simulink model "BMS_Protection_SoC"  (R2026b)
settings: Solver=VariableStepAuto
libraries: simulink x2
settings Model: Creator=maryliya  LastModifiedBy=maryliya

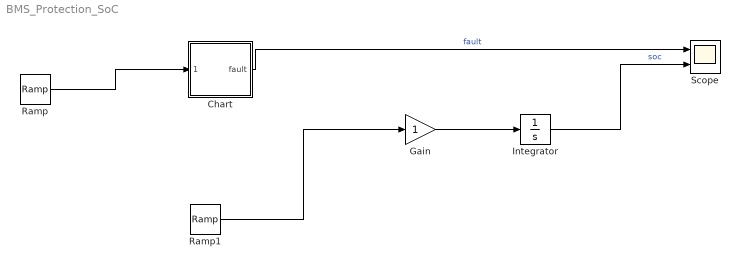
== system BMS_Protection_SoC ==
  Chart : Stateflow chart  TreatAsAtomicUnit=on
  Gain : Gain
  Integrator : Integrator
  Ramp : simulink/Sources/Ramp  slope=0.2  start=0  InitialOutput=2.8
  Ramp1 : simulink/Sources/Ramp  slope=1  start=0  InitialOutput=0
  Scope : Scope  NumInputPorts=2
      settings: ActiveDisplayYMinimum=-6.2500000000000027  ActiveDisplayYMaximum=56.250000000000043
  wires:
  Ramp1/1 -> Gain/1
  Gain/1 -> Integrator/1
  Ramp/1 -> Chart/1(voltage)
  Integrator/1 -> Scope/2  "soc"
  Chart/1(fault) -> Scope/1  "fault"

== stateflow chart BMS_Protection_SoC/Chart ==
  state Normal
    fault=0
  state OverVoltage_Fault
    fault=1
  state UnderVoltage_Fault
    fault=2
  Normal -> OverVoltage_Fault [order 1] : [voltage>4.2]
  OverVoltage_Fault -> Normal : [voltage<=4.2]
  (default) -> Normal
  Normal -> UnderVoltage_Fault [order 2] : [voltage<3.0]
  UnderVoltage_Fault -> Normal : [voltage>=3.0]
  data: voltage input; fault output
